simulink model "Drone_swarm_control"  (R2025a)
settings: Solver=FixedStepAuto  StartTime=0.0  StopTime=180  FixedStep=0.001  RelTol=1e-3
InitFcn:
  | %% Simulation parameters and waypoint trajectory
  | % Initial drone positions.
  | init_0=[0;0;0];
  | d_s=4;
  | init_1=init_0+d_s*[-1.1;0.1;0];
  | init_2=init_0+d_s*[0.3;-1.5;0];
  | init_3=init_0+d_s*[1.6;0.4;0];
  | init_4=init_0+d_s*[0.2;1.8;0];
  | 
  | % Initial battery energy in Wh.
  | E_0=77;
  | gain_2=1;
  | 
  | % PID controller gains.
  | PID_p=20;
  | PID_i=50;
  | PID_d=0;
  | 
  | % Router queues and background traffic.
  | router_buffer=160;
  | router_bandwith=300;
  | router_init_queue=[20,0,0,0,0];
  | traffic_mean=20;
  | traffic_variance=1;
  | 
  | % Communication-rate parameters.
  | F_max=2;
  | F_min=0.5;
  | F_H=(F_max+F_min)/3;
  | P_nc=(1-(F_H-F_min)/F_max);
  | 
  | 
  | % Desired formation offsets.
  | init_f_0=[0;0;0];
  | d_f=10;
  | init_f_1=init_0+d_f*[-1;0;0];
  | init_f_2=init_0+d_f*[0;-1;0];
  | init_f_3=init_0+d_f*[1;0;0];
  | init_f_4=init_0+d_f*[0;1;0];
  | 
  | 
  | % Waypoint mission with a fixed cruise altitude.
  | quota_fissa = -20;
  | 
  | waypoints = [
  |       0   0   0   0;
  |      75   0   quota_fissa   0;
  |     150   0   quota_fissa   0;
  |     225   0   quota_fissa   0;
  |     300   0   quota_fissa   0;
  |     300   0   quota_fissa   0;
  |     225  75   quota_fissa   0;
  |     150 150   quota_fissa   0;
  |      75 225   quota_fissa   0;
  |       0 300   quota_fissa   0;
  |       0 300   quota_fissa   0;
  |      75 300   quota_fissa   0;
  |     150 300   quota_fissa   0;
  |     225 300   quota_fissa   0;
  |     300 300   quota_fissa   0;
  | ... (+79 lines)
undefined symbols (not defined in the file): A_diacenza, DiscIntNeverNeededParam, L
libraries: dspsigops x10, robotcorelib x5, slpidlib x5, dspstat3 x5, simulink x1, uavutilslib x1
(part 3 of 4)

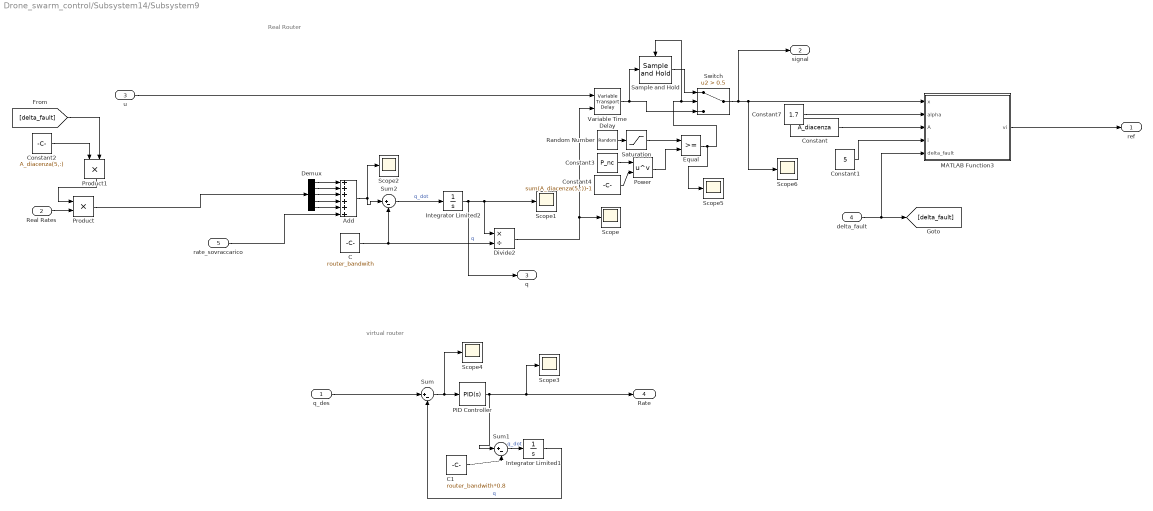
== system Drone_swarm_control/Subsystem14/Subsystem9 ==
  note: Real Router
  note: virtual router
  q_des : Inport
  " Real Rates" : Inport  Port=2
  u : Inport  Port=3
  delta_fault : Inport  Port=4
  "rate_sovraccarico " : Inport  Port=5
  Add : Sum  Inputs=++++++
  C : Constant  Value=router_bandwith
  C1 : Constant  Value=router_bandwith*0.8
  Constant : Constant  Value=A_diacenza
  Constant1 : Constant  Value=5
  Constant2 : Constant  Value=A_diacenza(5,:)
  Constant3 : Constant  Value=P_nc
  Constant4 : Constant  Value=sum(A_diacenza(5,:))-1
  Constant7 : Constant  Value=1.7
  Demux : Demux  Outputs=5
  Divide2 : Product  Inputs=*/
  Equal : RelationalOperator  OutDataTypeStr=boolean  RndMeth=Simplest  InputSameDT=off
  Integrator Limited1 : Integrator  InitialCondition=router_init_queue(1)  LimitOutput=on  UpperSaturationLimit=router_buffer  LowerSaturationLimit=0
  Integrator Limited2 : Integrator  InitialCondition=router_init_queue(5)  LimitOutput=on  UpperSaturationLimit=router_buffer  LowerSaturationLimit=0
  MATLAB Function3 : MATLAB Function  TreatAsAtomicUnit=on
  PID Controller : slpidlib/PID Controller  Controller=PID  Form=Parallel  TimeDomain=Continuous-time  UseExternalTs=off  SampleTime=-1  IntegratorMethod=Forward Euler  FilterMethod=Forward Euler  ControllerParametersSource=internal  P=PID_p  I=PID_i  UseKiTs=off  D=PID_d  UseExternalDerivativeSource=off  N=100  UseFilter=on  TunerSelectOption=Transfer Function Based (PID Tuner App)  InitialConditionSource=internal  InitialConditionForIntegrator=0  InitialConditionForFilter=0  DifferentiatorICPrevScaledInput=0  ExternalReset=none  TrackingMode=off  Kt=1  LimitOutput=off  SatLimitsSource=internal  UpperSaturationLimit=inf  LowerSaturationLimit=-inf  LinearizeAsGain=on  AntiWindupMode=none  Kb=1  LimitIntegrator=off  UpperIntegratorSaturationLimit=inf  LowerIntegratorSaturationLimit=-inf  POutMin=[]  POutMax=[]  IOutMin=[]  IOutMax=[]  DOutMin=[]  DOutMax=[]  NOutMin=[]  NOutMax=[]  SumOutMin=[]  SumOutMax=[]  SaturationOutMin=[]  SaturationOutMax=[]  PParamMin=[]  PParamMax=[]  IParamMin=[]  IParamMax=[]  DParamMin=[]  DParamMax=[]  NParamMin=[]  NParamMax=[]  KbParamMin=[]  KbParamMax=[]  KtParamMin=[]  KtParamMax=[]  KbOutMin=[]  KbOutMax=[]  KtOutMin=[]  KtOutMax=[]  IntegratorOutMin=[]  IntegratorOutMax=[]  FilterOutMin=[]  FilterOutMax=[]  SumI1OutMin=[]  SumI1OutMax=[]  SumI2OutMin=[]  SumI2OutMax=[]  SumI3OutMin=[]  SumI3OutMax=[]  SumI4OutMin=[]  SumI4OutMax=[]  SumDOutMin=[]  SumDOutMax=[]  DifferentiatorOutMin=[]  DifferentiatorOutMax=[]  FilterDiffOutCoefMin=[]  FilterDiffOutCoefMax=[]  ReciprocalOutMin=[]  ReciprocalOutMax=[]  SumDenOutMin=[]  SumDenOutMax=[]  SumNumOutMin=[]  SumNumOutMax=[]  DivideOutMin=[]  DivideOutMax=[]  UdiffTsProdOutMin=[]  UdiffTsProdOutMax=[]  NTsProdOutMin=[]  NTsProdOutMax=[]  UintegralTsProdOutMin=[]  UintegralTsProdOutMax=[]  UngainTsProdOutMin=[]  UngainTsProdOutMax=[]  ClampingZeroOutDataTypeStr=Inherit: Inherit via back propagation  ClampingZeroOutMin=[]  ClampingZeroOutMax=[]  FilterDenConstantOutDataTypeStr=Inherit: Inherit via back propagation  FilterDenConstantOutMin=[]  FilterDenConstantOutMax=[]  PCopyOutDataTypeStr=Inherit: Inherit via back propagation  PCopyOutMin=[]  PCopyOutMax=[]  NCopyOutDataTypeStr=Inherit: Inherit via back propagation  NCopyOutMin=[]  NCopyOutMax=[]  IntegratorContinuousStateAttributes=''  IntegratorStateMustResolveToSignalObject=off  IntegratorRTWStateStorageClass=Auto  FilterContinuousStateAttributes=''  FilterStateMustResolveToSignalObject=off  FilterRTWStateStorageClass=Auto  ParallelPVariant=InternalParameters  IdealPVariant=Disabled  IVariant=InternalParameters  DVariant=InternalParameters  IntegratorVariant=Continuous  SatVariant=Disabled  AWVariant=Passthrough  PCopyVariant=Disabled  TRVariant=Disabled  FdbkBlocksVariant=Forward  IdealPFdbkVariant=Disabled  SatFdbkVariant=Disabled  DerivativeFilterVariant=ContFilter  NVariant=InternalParameters  NCopyVariant=Disabled  FilterICVariant=InternalICsFilter  IntegratorICVariant=InternalICs  ExternalResetVariant=Disabled  TRSumVariant=Passthrough  SumFdbkVariant=Disabled  SumVariant=Sum_PID  TsampFilterVariant=InternalTs  TsampNgainVariant=Passthrough  TsampIntegralVariant=Disabled_SignalSpec  ExternalSaturationOutDataTypeStr=Inherit: Same as second input  DerivativeSourceVariant=ErrorSignal  PreIntVariant=InternalPreInt
  Power : Math  Operator=pow
  Product : Product
  Product1 : Product
  Random Number : RandomNumber  Mean=0.5  Variance=0.5  SampleTime=0.1
  Sample and Hold : dspsigops/Sample and Hold  trig=Rising edge  initCond=0  latchinput=off
  Saturation : Saturate  UpperLimit=1  LowerLimit=0
  Scope{,1..6} (7 alike) : Scope
      Scope settings: ActiveDisplayYMinimum=0.0019171133278549479  ActiveDisplayYMaximum=0.066506482659169808  DataLoggingVariableName=ScopeData7
      Scope1 settings: ActiveDisplayYMinimum=-1  ActiveDisplayYMaximum=1  DataLoggingVariableName=ScopeData8
      Scope2 settings: ActiveDisplayYMinimum=16.645701165470911  ActiveDisplayYMaximum=16.711897993083294  DataLoggingVariableName=ScopeData13
      Scope3 settings: ActiveDisplayYMinimum=-48.354575152001026  ActiveDisplayYMaximum=35.191176368009216  DataLoggingVariableName=ScopeData20
      Scope4 settings: ActiveDisplayYMinimum=-3.625  ActiveDisplayYMaximum=2.625  DataLoggingVariableName=ScopeData21
      Scope5 settings: ActiveDisplayYMinimum=-1  ActiveDisplayYMaximum=1  DataLoggingVariableName=ScopeData6
      Scope6 settings: ActiveDisplayYMinimum=-1  ActiveDisplayYMaximum=1  DataLoggingVariableName=ScopeData31
  Sum : Sum  Inputs=|+-
  Sum1 : Sum  Inputs=|+-
  Sum2 : Sum  Inputs=|+-
  Switch : Switch  Criteria=u2 > Threshold  Threshold=0.5  SaturateOnIntegerOverflow=off  InputSameDT=off
  Variable Time Delay : VariableTransportDelay  MaximumDelay=1000  InitialOutput=[init_0;zeros(6,1);init_1;zeros(6,1);init_2;zeros(6,1);init_3;zeros(6,1);init_4;zeros(6,1);]  MaximumPoints=1e4  ZeroDelay=on
  ref : Outport
  "signal " : Outport  Port=2
  q : Outport  Port=3
  " Rate" : Outport  Port=4
  wires:
  Constant7/1 -> MATLAB Function3/2(alpha)
  Constant/1 -> MATLAB Function3/3(A)
  Constant1/1 -> MATLAB Function3/4(i)
  MATLAB Function3/1(vi) -> ref/1
  Integrator Limited2/1 -> Scope1/1, Divide2/1, q/1  "q"
  Switch/1 -> "signal "/1, Scope6/1, MATLAB Function3/1(x)
  u/1 -> Variable Time Delay/1
  Sum2/1 -> Integrator Limited2/1  "q_dot"
  Divide2/1 -> Scope/1, Variable Time Delay/2
  C/1 -> Divide2/2, Sum2/2
  Sample and Hold/1 -> Switch/1
  Add/1 -> Sum2/1, Scope2/1
  Integrator Limited1/1 -> Sum/2  "q"
  PID Controller/1 -> Sum1/1, " Rate"/1, Scope3/1
  Sum1/1 -> Integrator Limited1/1  "q_dot"
  C1/1 -> Sum1/2
  Sum/1 -> Scope4/1, PID Controller/1
  q_des/1 -> Sum/1
  Demux/1 -> Add/1
  Demux/2 -> Add/2
  Demux/3 -> Add/3
  Demux/4 -> Add/4
  Demux/5 -> Add/5
  Power/1 -> Equal/2
  Saturation/1 -> Equal/1
  Random Number/1 -> Saturation/1
  Constant4/1 -> Power/2
  Equal/1 -> Scope5/1, Sample and Hold/Trigger, Switch/2
  Constant3/1 -> Power/1
  Variable Time Delay/1 -> Sample and Hold/1, Switch/3
  delta_fault/1 -> [delta_fault], MATLAB Function3/5(delta_fault)
  Product1/1 -> Product/1
  [delta_fault] -> Product1/2
  Constant2/1 -> Product1/1
  " Real Rates"/1 -> Product/2
  Product/1 -> Demux/1
  "rate_sovraccarico "/1 -> Add/6

== system Drone_swarm_control/Subsystem5/Subsystem ==
  output : Inport
  Cast To Double : DataTypeConversion  OutDataTypeStr=double  SaturateOnIntegerOverflow=off  RndMeth=Floor
  Constant : Constant  Value=5
  Constant1 : Constant
  Detect Rise Positive : simulink/Logic and Bit Operations/Detect Rise Positive  vinit=0  OutDataTypeStr=boolean
  Gain : Gain  Gain=1e5
  Integrator : Integrator  ExternalReset=rising
  Saturation : Saturate  UpperLimit=1  LowerLimit=0
  Scope{,1..3} (4 alike) : Scope
      Scope settings: ActiveDisplayYMinimum=-0.12499999999999997  ActiveDisplayYMaximum=1.125  DataLoggingVariableName=ScopeData46
      Scope1 settings: ActiveDisplayYMinimum=-1  ActiveDisplayYMaximum=1  DataLoggingVariableName=ScopeData47
      Scope2 settings: ActiveDisplayYMinimum=-0.00012499999999999998  ActiveDisplayYMaximum=0.0011250000000000001  DataLoggingVariableName=ScopeData48
      Scope3 settings: DataLoggingVariableName=ScopeData49
  Variable Transport Delay : VariableTransportDelay  MaximumDelay=10
  Variable Transport Delay1 : VariableTransportDelay  MaximumDelay=10
  Out1 : Outport
  wires:
  Variable Transport Delay/1 -> Scope1/1, Integrator/2
  Cast To Double/1 -> Integrator/1, Variable Transport Delay/1
  Integrator/1 -> Scope2/1, Gain/1
  Constant/1 -> Variable Transport Delay/2
  Saturation/1 -> Scope3/1, Out1/1
  output/1 -> Variable Transport Delay1/1
  Gain/1 -> Saturation/1
  Detect Rise Positive/1 -> Scope/1, Cast To Double/1
  Variable Transport Delay1/1 -> Detect Rise Positive/1
  Constant1/1 -> Variable Transport Delay1/2

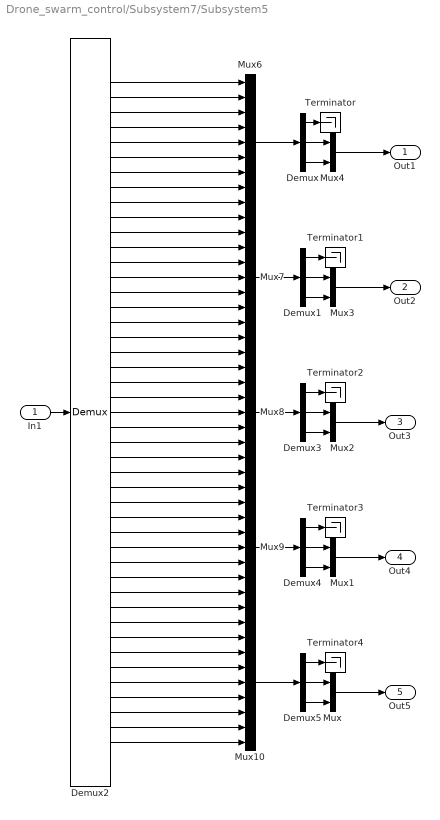
== system Drone_swarm_control/Subsystem7/Subsystem5 ==
  In1 : Inport
  Demux{,1,3..5} (5 alike) : Demux  Outputs=3
  Demux2 : Demux  Outputs=45
  Mux{,1..4} (5 alike) : Mux  Inputs=2
  Mux{6..10} (5 alike) : Mux  Inputs=9
  Terminator{,1..4} (5 alike) : Terminator
  Out1 : Outport
  Out2 : Outport  Port=2
  Out3 : Outport  Port=3
  Out4 : Outport  Port=4
  Out5 : Outport  Port=5
  wires:
  Demux2/4 -> Mux6/4
  Demux2/22 -> Mux8/4
  Demux2/7 -> Mux6/7
  Demux2/5 -> Mux6/5
  Demux2/37 -> Mux10/1
  Demux2/32 -> Mux9/5
  Demux2/11 -> Mux7/2
  Demux2/35 -> Mux9/8
  Demux2/39 -> Mux10/3
  Demux2/12 -> Mux7/3
  Demux2/9 -> Mux6/9
  Demux2/18 -> Mux7/9
  Demux2/25 -> Mux8/7
  Demux2/6 -> Mux6/6
  Demux2/31 -> Mux9/4
  Demux2/42 -> Mux10/6
  Demux2/1 -> Mux6/1
  Demux2/17 -> Mux7/8
  Demux2/29 -> Mux9/2
  Demux2/24 -> Mux8/6
  Demux2/8 -> Mux6/8
  Demux2/28 -> Mux9/1
  Demux2/45 -> Mux10/9
  Demux2/44 -> Mux10/8
  Demux2/16 -> Mux7/7
  Demux2/38 -> Mux10/2
  Demux2/21 -> Mux8/3
  Demux2/19 -> Mux8/1
  Demux2/33 -> Mux9/6
  Demux2/36 -> Mux9/9
  Demux2/23 -> Mux8/5
  Demux2/43 -> Mux10/7
  Demux2/30 -> Mux9/3
  Demux2/41 -> Mux10/5
  Demux2/34 -> Mux9/7
  Demux2/14 -> Mux7/5
  Demux2/15 -> Mux7/6
  Demux2/3 -> Mux6/3
  Demux2/13 -> Mux7/4
  Demux2/26 -> Mux8/8
  Demux2/20 -> Mux8/2
  Demux2/2 -> Mux6/2
  Demux2/27 -> Mux8/9
  Demux2/10 -> Mux7/1
  Demux2/40 -> Mux10/4
  In1/1 -> Demux2/1
  Mux6/1 -> Demux/1
  Mux7/1 -> Demux1/1
  Mux8/1 -> Demux3/1
  Mux9/1 -> Demux4/1
  Mux10/1 -> Demux5/1
  Demux/1 -> Terminator/1
  Demux1/1 -> Terminator1/1
  Demux3/1 -> Terminator2/1
  Demux4/1 -> Terminator3/1
  Demux5/1 -> Terminator4/1
  Demux5/3 -> Mux/2
  Demux5/2 -> Mux/1
  Mux/1 -> Out5/1
  Demux4/2 -> Mux1/1
  Demux4/3 -> Mux1/2
  Mux1/1 -> Out4/1
  Demux3/2 -> Mux2/1
  Demux3/3 -> Mux2/2
  Mux2/1 -> Out3/1
  Demux1/2 -> Mux3/1
  Demux1/3 -> Mux3/2
  Mux3/1 -> Out2/1
  Demux/2 -> Mux4/1
  Demux/3 -> Mux4/2
  Mux4/1 -> Out1/1

== system Drone_swarm_control/trasmission/Subsystem1 ==
  note: Subsystem13
  In : Inport
  In1 : Inport  Port=2
  Constant13 : Constant
  Constant2 : Constant
  Divide : Product  Inputs=*/
  Integrator : Integrator  ExternalReset=rising
  Relational Operator : RelationalOperator  Operator=<=  OutDataTypeStr=boolean  RndMeth=Simplest  InputSameDT=off
  Sample and Hold5 : dspsigops/Sample and Hold  trig=Rising edge  initCond=0  latchinput=off
  Scope3 : Scope
      settings: ActiveDisplayYMinimum=-3.131696080231905E+7  ActiveDisplayYMaximum=3.596063759040764E+7  DataLoggingVariableName=ScopeData9
  Switch : Switch  Criteria=u2 > Threshold  SaturateOnIntegerOverflow=off  InputSameDT=off
  Unit Delay : UnitDelay  SampleTime=Ts  HasFrameUpgradeWarning=on
  " " : Outport
  wires:
  In/1 -> Sample and Hold5/1
  Constant2/1 -> Integrator/1
  In1/1 -> Divide/2
  Unit Delay/1 -> Integrator/2
  Constant13/1 -> Divide/1
  Divide/1 -> Relational Operator/1, Scope3/1
  Relational Operator/1 -> Unit Delay/1, Sample and Hold5/Trigger
  Sample and Hold5/1 -> " "/1
  Integrator/1 -> Relational Operator/2

== system Drone_swarm_control/trasmission/Subsystem2 ==
  note: Subsystem13
  In : Inport
  In1 : Inport  Port=2
  Constant13 : Constant
  Constant2 : Constant
  Divide : Product  Inputs=*/
  Integrator : Integrator  ExternalReset=rising
  Relational Operator : RelationalOperator  Operator=<=  OutDataTypeStr=boolean  RndMeth=Simplest  InputSameDT=off
  Sample and Hold5 : dspsigops/Sample and Hold  trig=Rising edge  initCond=0  latchinput=off
  Scope3 : Scope
      settings: ActiveDisplayYMinimum=-3.131696080231905E+7  ActiveDisplayYMaximum=3.596063759040764E+7  DataLoggingVariableName=ScopeData9
  Unit Delay : UnitDelay  SampleTime=Ts  HasFrameUpgradeWarning=on
  " " : Outport
  wires:
  In/1 -> Sample and Hold5/1
  Constant2/1 -> Integrator/1
  In1/1 -> Divide/2
  Unit Delay/1 -> Integrator/2
  Constant13/1 -> Divide/1
  Divide/1 -> Relational Operator/1, Scope3/1
  Relational Operator/1 -> Unit Delay/1, Sample and Hold5/Trigger
  Sample and Hold5/1 -> " "/1
  Integrator/1 -> Relational Operator/2

== system Drone_swarm_control/trasmission/Subsystem3 ==
  note: Subsystem13
  In : Inport
  In1 : Inport  Port=2
  Constant13 : Constant
  Constant2 : Constant
  Divide : Product  Inputs=*/
  Integrator : Integrator  ExternalReset=rising
  Relational Operator : RelationalOperator  Operator=<=  OutDataTypeStr=boolean  RndMeth=Simplest  InputSameDT=off
  Sample and Hold5 : dspsigops/Sample and Hold  trig=Rising edge  initCond=0  latchinput=off
  Scope3 : Scope
      settings: ActiveDisplayYMinimum=-3.131696080231905E+7  ActiveDisplayYMaximum=3.596063759040764E+7  DataLoggingVariableName=ScopeData9
  Unit Delay : UnitDelay  SampleTime=Ts  HasFrameUpgradeWarning=on
  " " : Outport
  wires:
  Integrator/1 -> Relational Operator/2
  Sample and Hold5/1 -> " "/1
  Relational Operator/1 -> Sample and Hold5/Trigger, Unit Delay/1
  Divide/1 -> Scope3/1, Relational Operator/1
  Constant13/1 -> Divide/1
  Unit Delay/1 -> Integrator/2
  In1/1 -> Divide/2
  Constant2/1 -> Integrator/1
  In/1 -> Sample and Hold5/1

== system Drone_swarm_control/trasmission/Subsystem4 ==
  note: Subsystem13
  In : Inport
  In1 : Inport  Port=2
  Constant13 : Constant
  Constant2 : Constant
  Divide : Product  Inputs=*/
  Integrator : Integrator  ExternalReset=rising
  Relational Operator : RelationalOperator  Operator=<=  OutDataTypeStr=boolean  RndMeth=Simplest  InputSameDT=off
  Sample and Hold5 : dspsigops/Sample and Hold  trig=Rising edge  initCond=0  latchinput=off
  Scope3 : Scope
      settings: ActiveDisplayYMinimum=-3.131696080231905E+7  ActiveDisplayYMaximum=3.596063759040764E+7  DataLoggingVariableName=ScopeData9
  Unit Delay : UnitDelay  SampleTime=Ts  HasFrameUpgradeWarning=on
  " " : Outport
  wires:
  In/1 -> Sample and Hold5/1
  Constant2/1 -> Integrator/1
  In1/1 -> Divide/2
  Unit Delay/1 -> Integrator/2
  Constant13/1 -> Divide/1
  Divide/1 -> Relational Operator/1, Scope3/1
  Relational Operator/1 -> Unit Delay/1, Sample and Hold5/Trigger
  Sample and Hold5/1 -> " "/1
  Integrator/1 -> Relational Operator/2

== system Drone_swarm_control/trasmission/Subsystem5 ==
  note: Subsystem13
  In : Inport
  In1 : Inport  Port=2
  Constant13 : Constant
  Constant2 : Constant
  Divide : Product  Inputs=*/
  Integrator : Integrator  ExternalReset=rising
  Relational Operator : RelationalOperator  Operator=<=  OutDataTypeStr=boolean  RndMeth=Simplest  InputSameDT=off
  Sample and Hold5 : dspsigops/Sample and Hold  trig=Rising edge  initCond=0  latchinput=off
  Scope3 : Scope
      settings: ActiveDisplayYMinimum=-3.131696080231905E+7  ActiveDisplayYMaximum=3.596063759040764E+7  DataLoggingVariableName=ScopeData9
  Unit Delay : UnitDelay  SampleTime=Ts  HasFrameUpgradeWarning=on
  " " : Outport
  wires:
  Integrator/1 -> Relational Operator/2
  Sample and Hold5/1 -> " "/1
  Relational Operator/1 -> Sample and Hold5/Trigger, Unit Delay/1
  Divide/1 -> Scope3/1, Relational Operator/1
  Constant13/1 -> Divide/1
  Unit Delay/1 -> Integrator/2
  In1/1 -> Divide/2
  Constant2/1 -> Integrator/1
  In/1 -> Sample and Hold5/1

== system Drone_swarm_control/trasmission/rate_min ==
  r_req : Inport
  delta_fault : Inport  Port=2
  Constant : Constant  Value=A_diacenza
  MATLAB Function : MATLAB Function  TreatAsAtomicUnit=on
  MATLAB Function1 : MATLAB Function  TreatAsAtomicUnit=on
  MATLAB Function2 : MATLAB Function  TreatAsAtomicUnit=on
  MATLAB Function3 : MATLAB Function  TreatAsAtomicUnit=on
  MATLAB Function4 : MATLAB Function  TreatAsAtomicUnit=on
  MATLAB Function5 : MATLAB Function  TreatAsAtomicUnit=on
  Minimum{,1..4} (5 alike) : dspstat3/Minimum  operation=minimum  fcn=Value  indexBase=One  operateOver=Each column  Dimension=1  InputProcessing=Columns as channels (frame based)  reset=None  roiEnable=off  roiType=Rectangles  roiPortion=Entire ROI  roiOutput=Individual statistics for each ROI  roiFlag=off  roundingMode=Floor  overflowMode=off
      settings: LibrarySourceBlock=dsphdlsupportstat/Minimum
  Mux1 : Mux  Inputs=5
  Product{,1..4} (5 alike) : Product
  r_min : Outport
  wires:
  MATLAB Function/1(y) -> Minimum/1
  Minimum3/1 -> Mux1/4
  Mux1/1 -> r_min/1
  MATLAB Function4/1(y) -> Minimum4/1
  Minimum2/1 -> Mux1/3
  Minimum4/1 -> Mux1/5
  MATLAB Function2/1(y) -> Minimum2/1
  MATLAB Function1/1(y) -> Minimum1/1
  Minimum/1 -> Mux1/1
  Minimum1/1 -> Mux1/2
  MATLAB Function3/1(y) -> Minimum3/1
  delta_fault/1 -> MATLAB Function5/2(delta)
  Constant/1 -> MATLAB Function5/1(A)
  Product/1 -> MATLAB Function/1(u)
  Product1/1 -> MATLAB Function1/1(u)
  Product2/1 -> MATLAB Function2/1(u)
  Product3/1 -> MATLAB Function3/1(u)
  Product4/1 -> MATLAB Function4/1(u)
  r_req/1 -> Product1/2, Product/2, Product4/2, Product3/2, Product2/2
  MATLAB Function5/1(A_edit1) -> Product/1
  MATLAB Function5/2(A_edit2) -> Product1/1
  MATLAB Function5/3(A_edit3) -> Product2/1
  MATLAB Function5/4(A_edit4) -> Product3/1
  MATLAB Function5/5(A_edit5) -> Product4/1

== system Drone_swarm_control/Subsystem1/Subsystem_1/Inner-loop control ==
  zb_des : Inport
  Rb : Inport  Port=2
  omega_bb : Inport  Port=3
  xb_des : Inport  Port=4
  Derivation : DiscreteTransferFcn  Numerator=[1 -1]  Denominator=[Ts 0]  InitialStates=[1 0 0;0 1 0;0 0 1]  SampleTime=Ts
  Derivation1 : DiscreteTransferFcn  Numerator=[1 -1]  Denominator=[Ts 0]  InitialStates=[0 0 0]  SampleTime=Ts
  Inner-loop control : MATLAB Function  TreatAsAtomicUnit=on
  Unit Delay1 : UnitDelay  InitialCondition=eye(3)  SampleTime=Ts
  Unit Delay3 : UnitDelay  InitialCondition=[0 0 0]  SampleTime=Ts
  tau : Outport
  err_R : Outport  Port=2
  err_W : Outport  Port=3
  wires:
  Inner-loop control/2(omega_bb_des) -> Derivation1/1
  Inner-loop control/1(Rb_des) -> Derivation/1
  omega_bb/1 -> Inner-loop control/4(omega_bb)
  zb_des/1 -> Inner-loop control/1(zb_des)
  Derivation/1 -> Unit Delay1/1
  Unit Delay3/1 -> Inner-loop control/5(dot_omega_bb_des)
  Inner-loop control/5(err_W) -> err_W/1
  Derivation1/1 -> Unit Delay3/1
  Unit Delay1/1 -> Inner-loop control/3(dot_Rb_des)
  Inner-loop control/3(tau) -> tau/1
  Rb/1 -> Inner-loop control/2(Rb)
  Inner-loop control/4(err_R) -> err_R/1
  xb_des/1 -> Inner-loop control/6(xb_des)

== system Drone_swarm_control/Subsystem1/Subsystem_1/Planner ==
  References : Inport
  Constant : Constant  Value=0
  Demux : Demux  Outputs=10
  Mux{1..4} (4 alike) : Mux  Inputs=3
  Trigonometric Function : Trigonometry
  Trigonometric Function1 : Trigonometry  Operator=cos
  position_des : Outport
  linear_velocity_des : Outport  Port=2
  linear_acceleration_des : Outport  Port=3
  xb_des : Outport  Port=4
  wires:
  References/1 -> Demux/1
  Demux/10 -> Trigonometric Function1/1, Trigonometric Function/1
  Demux/9 -> Mux1/3
  Demux/8 -> Mux1/2
  Demux/7 -> Mux1/1
  Demux/6 -> Mux3/3
  Demux/5 -> Mux3/2
  Demux/4 -> Mux3/1
  Demux/3 -> Mux2/3
  Demux/2 -> Mux2/2
  Demux/1 -> Mux2/1
  Constant/1 -> Mux4/3
  Trigonometric Function1/1 -> Mux4/1
  Trigonometric Function/1 -> Mux4/2
  Mux4/1 -> xb_des/1
  Mux2/1 -> position_des/1
  Mux3/1 -> linear_velocity_des/1
  Mux1/1 -> linear_acceleration_des/1

== system Drone_swarm_control/Subsystem1/Subsystem_1/Quadrotor dynamics ==
  uT : Inport
  tau_b : Inport  Port=2
  Integrator : Integrator  InitialCondition=init_0
  Integrator1 : Integrator  InitialCondition=lin_vel_0
  Integrator2 : Integrator  InitialCondition=[1 0 0; 0 1 0;0 0 1]
  Integrator3 : Integrator  InitialCondition=w_bb_0
  MATLAB Function1 : MATLAB Function  TreatAsAtomicUnit=on
  UAV dynamics : MATLAB Function  TreatAsAtomicUnit=on
  Position : Outport
  Linear_velocity : Outport  Port=2
  Rb : Outport  Port=3
  dot_Rb : Outport  Port=4
  omega_bb : Outport  Port=5
  dot_omega_bb : Outport  Port=6
  lin_acc : Outport  Port=7
  wires:
  Integrator2/1 -> MATLAB Function1/1(Rb_temp)
  MATLAB Function1/1(Rb) -> UAV dynamics/3(Rb), Rb/1
  UAV dynamics/2(dot_Rb) -> dot_Rb/1, Integrator2/1
  Integrator3/1 -> UAV dynamics/4(omega_bb), omega_bb/1
  Integrator1/1 -> Integrator/1, Linear_velocity/1
  uT/1 -> UAV dynamics/1(uT)
  UAV dynamics/1(lin_acc) -> Integrator1/1, lin_acc/1
  UAV dynamics/3(ang_acc) -> Integrator3/1, dot_omega_bb/1
  Integrator/1 -> Position/1
  tau_b/1 -> UAV dynamics/2(tau_b)

== system Drone_swarm_control/Subsystem1/Subsystem_2/Inner-loop control ==
  zb_des : Inport
  Rb : Inport  Port=2
  omega_bb : Inport  Port=3
  xb_des : Inport  Port=4
  Derivation : DiscreteTransferFcn  Numerator=[1 -1]  Denominator=[Ts 0]  InitialStates=[1 0 0;0 1 0;0 0 1]  SampleTime=Ts
  Derivation1 : DiscreteTransferFcn  Numerator=[1 -1]  Denominator=[Ts 0]  InitialStates=[0 0 0]  SampleTime=Ts
  Inner-loop control : MATLAB Function  TreatAsAtomicUnit=on
  Unit Delay1 : UnitDelay  InitialCondition=eye(3)  SampleTime=Ts
  Unit Delay3 : UnitDelay  InitialCondition=[0 0 0]  SampleTime=Ts
  tau : Outport
  err_R : Outport  Port=2
  err_W : Outport  Port=3
  wires:
  Inner-loop control/2(omega_bb_des) -> Derivation1/1
  Inner-loop control/1(Rb_des) -> Derivation/1
  omega_bb/1 -> Inner-loop control/4(omega_bb)
  zb_des/1 -> Inner-loop control/1(zb_des)
  Derivation/1 -> Unit Delay1/1
  Unit Delay3/1 -> Inner-loop control/5(dot_omega_bb_des)
  Inner-loop control/5(err_W) -> err_W/1
  Derivation1/1 -> Unit Delay3/1
  Unit Delay1/1 -> Inner-loop control/3(dot_Rb_des)
  Inner-loop control/3(tau) -> tau/1
  Rb/1 -> Inner-loop control/2(Rb)
  Inner-loop control/4(err_R) -> err_R/1
  xb_des/1 -> Inner-loop control/6(xb_des)

== system Drone_swarm_control/Subsystem1/Subsystem_2/Planner ==
  References : Inport
  Constant : Constant  Value=0
  Demux : Demux  Outputs=10
  Mux{1..4} (4 alike) : Mux  Inputs=3
  Trigonometric Function : Trigonometry
  Trigonometric Function1 : Trigonometry  Operator=cos
  position_des : Outport
  linear_velocity_des : Outport  Port=2
  linear_acceleration_des : Outport  Port=3
  xb_des : Outport  Port=4
  wires:
  References/1 -> Demux/1
  Demux/10 -> Trigonometric Function1/1, Trigonometric Function/1
  Demux/9 -> Mux1/3
  Demux/8 -> Mux1/2
  Demux/7 -> Mux1/1
  Demux/6 -> Mux3/3
  Demux/5 -> Mux3/2
  Demux/4 -> Mux3/1
  Demux/3 -> Mux2/3
  Demux/2 -> Mux2/2
  Demux/1 -> Mux2/1
  Constant/1 -> Mux4/3
  Trigonometric Function1/1 -> Mux4/1
  Trigonometric Function/1 -> Mux4/2
  Mux4/1 -> xb_des/1
  Mux2/1 -> position_des/1
  Mux3/1 -> linear_velocity_des/1
  Mux1/1 -> linear_acceleration_des/1

== system Drone_swarm_control/Subsystem1/Subsystem_2/Quadrotor dynamics ==
  uT : Inport
  tau_b : Inport  Port=2
  Integrator : Integrator  InitialCondition=init_1
  Integrator1 : Integrator  InitialCondition=lin_vel_0
  Integrator2 : Integrator  InitialCondition=[1 0 0; 0 1 0;0 0 1]
  Integrator3 : Integrator  InitialCondition=w_bb_0
  MATLAB Function1 : MATLAB Function  TreatAsAtomicUnit=on
  UAV dynamics : MATLAB Function  TreatAsAtomicUnit=on
  Position : Outport
  Linear_velocity : Outport  Port=2
  Rb : Outport  Port=3
  dot_Rb : Outport  Port=4
  omega_bb : Outport  Port=5
  dot_omega_bb : Outport  Port=6
  lin_acc : Outport  Port=7
  wires:
  Integrator2/1 -> MATLAB Function1/1(Rb_temp)
  MATLAB Function1/1(Rb) -> UAV dynamics/3(Rb), Rb/1
  UAV dynamics/2(dot_Rb) -> dot_Rb/1, Integrator2/1
  Integrator3/1 -> omega_bb/1, UAV dynamics/4(omega_bb)
  Integrator1/1 -> Integrator/1, Linear_velocity/1
  uT/1 -> UAV dynamics/1(uT)
  UAV dynamics/1(lin_acc) -> Integrator1/1, lin_acc/1
  UAV dynamics/3(ang_acc) -> Integrator3/1, dot_omega_bb/1
  Integrator/1 -> Position/1
  tau_b/1 -> UAV dynamics/2(tau_b)

== system Drone_swarm_control/Subsystem1/Subsystem_3/Inner-loop control ==
  zb_des : Inport
  Rb : Inport  Port=2
  omega_bb : Inport  Port=3
  xb_des : Inport  Port=4
  Derivation : DiscreteTransferFcn  Numerator=[1 -1]  Denominator=[Ts 0]  InitialStates=[1 0 0;0 1 0;0 0 1]  SampleTime=Ts
  Derivation1 : DiscreteTransferFcn  Numerator=[1 -1]  Denominator=[Ts 0]  InitialStates=[0 0 0]  SampleTime=Ts
  Inner-loop control : MATLAB Function  TreatAsAtomicUnit=on
  Unit Delay1 : UnitDelay  InitialCondition=eye(3)  SampleTime=Ts
  Unit Delay3 : UnitDelay  InitialCondition=[0 0 0]  SampleTime=Ts
  tau : Outport
  err_R : Outport  Port=2
  err_W : Outport  Port=3
  wires:
  Inner-loop control/2(omega_bb_des) -> Derivation1/1
  Inner-loop control/1(Rb_des) -> Derivation/1
  omega_bb/1 -> Inner-loop control/4(omega_bb)
  zb_des/1 -> Inner-loop control/1(zb_des)
  Derivation/1 -> Unit Delay1/1
  Unit Delay3/1 -> Inner-loop control/5(dot_omega_bb_des)
  Inner-loop control/5(err_W) -> err_W/1
  Derivation1/1 -> Unit Delay3/1
  Unit Delay1/1 -> Inner-loop control/3(dot_Rb_des)
  Inner-loop control/3(tau) -> tau/1
  Rb/1 -> Inner-loop control/2(Rb)
  Inner-loop control/4(err_R) -> err_R/1
  xb_des/1 -> Inner-loop control/6(xb_des)

== system Drone_swarm_control/Subsystem1/Subsystem_3/Planner ==
  References : Inport
  Constant : Constant  Value=0
  Demux : Demux  Outputs=10
  Mux{1..4} (4 alike) : Mux  Inputs=3
  Trigonometric Function : Trigonometry
  Trigonometric Function1 : Trigonometry  Operator=cos
  position_des : Outport
  linear_velocity_des : Outport  Port=2
  linear_acceleration_des : Outport  Port=3
  xb_des : Outport  Port=4
  wires:
  References/1 -> Demux/1
  Demux/10 -> Trigonometric Function1/1, Trigonometric Function/1
  Demux/9 -> Mux1/3
  Demux/8 -> Mux1/2
  Demux/7 -> Mux1/1
  Demux/6 -> Mux3/3
  Demux/5 -> Mux3/2
  Demux/4 -> Mux3/1
  Demux/3 -> Mux2/3
  Demux/2 -> Mux2/2
  Demux/1 -> Mux2/1
  Constant/1 -> Mux4/3
  Trigonometric Function1/1 -> Mux4/1
  Trigonometric Function/1 -> Mux4/2
  Mux4/1 -> xb_des/1
  Mux2/1 -> position_des/1
  Mux3/1 -> linear_velocity_des/1
  Mux1/1 -> linear_acceleration_des/1

== system Drone_swarm_control/Subsystem1/Subsystem_3/Quadrotor dynamics ==
  uT : Inport
  tau_b : Inport  Port=2
  Integrator : Integrator  InitialCondition=init_2
  Integrator1 : Integrator  InitialCondition=lin_vel_0
  Integrator2 : Integrator  InitialCondition=[1 0 0; 0 1 0;0 0 1]
  Integrator3 : Integrator  InitialCondition=w_bb_0
  MATLAB Function1 : MATLAB Function  TreatAsAtomicUnit=on
  UAV dynamics : MATLAB Function  TreatAsAtomicUnit=on
  Position : Outport
  Linear_velocity : Outport  Port=2
  Rb : Outport  Port=3
  dot_Rb : Outport  Port=4
  omega_bb : Outport  Port=5
  dot_omega_bb : Outport  Port=6
  lin_acc : Outport  Port=7
  wires:
  Integrator2/1 -> MATLAB Function1/1(Rb_temp)
  MATLAB Function1/1(Rb) -> UAV dynamics/3(Rb), Rb/1
  UAV dynamics/2(dot_Rb) -> dot_Rb/1, Integrator2/1
  Integrator3/1 -> omega_bb/1, UAV dynamics/4(omega_bb)
  Integrator1/1 -> Integrator/1, Linear_velocity/1
  uT/1 -> UAV dynamics/1(uT)
  UAV dynamics/1(lin_acc) -> Integrator1/1, lin_acc/1
  UAV dynamics/3(ang_acc) -> Integrator3/1, dot_omega_bb/1
  Integrator/1 -> Position/1
  tau_b/1 -> UAV dynamics/2(tau_b)

== system Drone_swarm_control/Subsystem1/Subsystem_4/Inner-loop control ==
  zb_des : Inport
  Rb : Inport  Port=2
  omega_bb : Inport  Port=3
  xb_des : Inport  Port=4
  Derivation : DiscreteTransferFcn  Numerator=[1 -1]  Denominator=[Ts 0]  InitialStates=[1 0 0;0 1 0;0 0 1]  SampleTime=Ts
  Derivation1 : DiscreteTransferFcn  Numerator=[1 -1]  Denominator=[Ts 0]  InitialStates=[0 0 0]  SampleTime=Ts
  Inner-loop control : MATLAB Function  TreatAsAtomicUnit=on
  Unit Delay1 : UnitDelay  InitialCondition=eye(3)  SampleTime=Ts
  Unit Delay3 : UnitDelay  InitialCondition=[0 0 0]  SampleTime=Ts
  tau : Outport
  err_R : Outport  Port=2
  err_W : Outport  Port=3
  wires:
  Inner-loop control/2(omega_bb_des) -> Derivation1/1
  Inner-loop control/1(Rb_des) -> Derivation/1
  omega_bb/1 -> Inner-loop control/4(omega_bb)
  zb_des/1 -> Inner-loop control/1(zb_des)
  Derivation/1 -> Unit Delay1/1
  Unit Delay3/1 -> Inner-loop control/5(dot_omega_bb_des)
  Inner-loop control/5(err_W) -> err_W/1
  Derivation1/1 -> Unit Delay3/1
  Unit Delay1/1 -> Inner-loop control/3(dot_Rb_des)
  Inner-loop control/3(tau) -> tau/1
  Rb/1 -> Inner-loop control/2(Rb)
  Inner-loop control/4(err_R) -> err_R/1
  xb_des/1 -> Inner-loop control/6(xb_des)

== system Drone_swarm_control/Subsystem1/Subsystem_4/Planner ==
  References : Inport
  Constant : Constant  Value=0
  Demux : Demux  Outputs=10
  Mux{1..4} (4 alike) : Mux  Inputs=3
  Trigonometric Function : Trigonometry
  Trigonometric Function1 : Trigonometry  Operator=cos
  position_des : Outport
  linear_velocity_des : Outport  Port=2
  linear_acceleration_des : Outport  Port=3
  xb_des : Outport  Port=4
  wires:
  References/1 -> Demux/1
  Demux/10 -> Trigonometric Function1/1, Trigonometric Function/1
  Demux/9 -> Mux1/3
  Demux/8 -> Mux1/2
  Demux/7 -> Mux1/1
  Demux/6 -> Mux3/3
  Demux/5 -> Mux3/2
  Demux/4 -> Mux3/1
  Demux/3 -> Mux2/3
  Demux/2 -> Mux2/2
  Demux/1 -> Mux2/1
  Constant/1 -> Mux4/3
  Trigonometric Function1/1 -> Mux4/1
  Trigonometric Function/1 -> Mux4/2
  Mux4/1 -> xb_des/1
  Mux2/1 -> position_des/1
  Mux1/1 -> linear_acceleration_des/1
  Mux3/1 -> linear_velocity_des/1

== system Drone_swarm_control/Subsystem1/Subsystem_4/Quadrotor dynamics ==
  uT : Inport
  tau_b : Inport  Port=2
  Integrator : Integrator  InitialCondition=init_3
  Integrator1 : Integrator  InitialCondition=lin_vel_0
  Integrator2 : Integrator  InitialCondition=[1 0 0; 0 1 0;0 0 1]
  Integrator3 : Integrator  InitialCondition=w_bb_0
  MATLAB Function1 : MATLAB Function  TreatAsAtomicUnit=on
  UAV dynamics : MATLAB Function  TreatAsAtomicUnit=on
  Position : Outport
  Linear_velocity : Outport  Port=2
  Rb : Outport  Port=3
  dot_Rb : Outport  Port=4
  omega_bb : Outport  Port=5
  dot_omega_bb : Outport  Port=6
  lin_acc : Outport  Port=7
  wires:
  Integrator2/1 -> MATLAB Function1/1(Rb_temp)
  MATLAB Function1/1(Rb) -> UAV dynamics/3(Rb), Rb/1
  UAV dynamics/2(dot_Rb) -> dot_Rb/1, Integrator2/1
  Integrator3/1 -> omega_bb/1, UAV dynamics/4(omega_bb)
  Integrator1/1 -> Integrator/1, Linear_velocity/1
  uT/1 -> UAV dynamics/1(uT)
  UAV dynamics/1(lin_acc) -> Integrator1/1, lin_acc/1
  UAV dynamics/3(ang_acc) -> Integrator3/1, dot_omega_bb/1
  Integrator/1 -> Position/1
  tau_b/1 -> UAV dynamics/2(tau_b)

== system Drone_swarm_control/Subsystem1/Subsystem_5/Inner-loop control ==
  zb_des : Inport
  Rb : Inport  Port=2
  omega_bb : Inport  Port=3
  xb_des : Inport  Port=4
  Derivation : DiscreteTransferFcn  Numerator=[1 -1]  Denominator=[Ts 0]  InitialStates=[1 0 0;0 1 0;0 0 1]  SampleTime=Ts
  Derivation1 : DiscreteTransferFcn  Numerator=[1 -1]  Denominator=[Ts 0]  InitialStates=[0 0 0]  SampleTime=Ts
  Inner-loop control : MATLAB Function  TreatAsAtomicUnit=on
  Unit Delay1 : UnitDelay  InitialCondition=eye(3)  SampleTime=Ts
  Unit Delay3 : UnitDelay  InitialCondition=[0 0 0]  SampleTime=Ts
  tau : Outport
  err_R : Outport  Port=2
  err_W : Outport  Port=3
  wires:
  Inner-loop control/2(omega_bb_des) -> Derivation1/1
  Inner-loop control/1(Rb_des) -> Derivation/1
  omega_bb/1 -> Inner-loop control/4(omega_bb)
  zb_des/1 -> Inner-loop control/1(zb_des)
  Derivation/1 -> Unit Delay1/1
  Unit Delay3/1 -> Inner-loop control/5(dot_omega_bb_des)
  Inner-loop control/5(err_W) -> err_W/1
  Derivation1/1 -> Unit Delay3/1
  Unit Delay1/1 -> Inner-loop control/3(dot_Rb_des)
  Inner-loop control/3(tau) -> tau/1
  Rb/1 -> Inner-loop control/2(Rb)
  Inner-loop control/4(err_R) -> err_R/1
  xb_des/1 -> Inner-loop control/6(xb_des)

== system Drone_swarm_control/Subsystem1/Subsystem_5/Planner ==
  References : Inport
  Constant : Constant  Value=0
  Demux : Demux  Outputs=10
  Mux{1..4} (4 alike) : Mux  Inputs=3
  Trigonometric Function : Trigonometry
  Trigonometric Function1 : Trigonometry  Operator=cos
  position_des : Outport
  linear_velocity_des : Outport  Port=2
  linear_acceleration_des : Outport  Port=3
  xb_des : Outport  Port=4
  wires:
  References/1 -> Demux/1
  Demux/10 -> Trigonometric Function1/1, Trigonometric Function/1
  Demux/9 -> Mux1/3
  Demux/8 -> Mux1/2
  Demux/7 -> Mux1/1
  Demux/6 -> Mux3/3
  Demux/5 -> Mux3/2
  Demux/4 -> Mux3/1
  Demux/3 -> Mux2/3
  Demux/2 -> Mux2/2
  Demux/1 -> Mux2/1
  Constant/1 -> Mux4/3
  Trigonometric Function1/1 -> Mux4/1
  Trigonometric Function/1 -> Mux4/2
  Mux4/1 -> xb_des/1
  Mux2/1 -> position_des/1
  Mux1/1 -> linear_acceleration_des/1
  Mux3/1 -> linear_velocity_des/1

== system Drone_swarm_control/Subsystem1/Subsystem_5/Quadrotor dynamics ==
  uT : Inport
  tau_b : Inport  Port=2
  Integrator : Integrator  InitialCondition=init_4
  Integrator1 : Integrator  InitialCondition=lin_vel_0
  Integrator2 : Integrator  InitialCondition=[1 0 0; 0 1 0;0 0 1]
  Integrator3 : Integrator  InitialCondition=w_bb_0
  MATLAB Function1 : MATLAB Function  TreatAsAtomicUnit=on
  UAV dynamics : MATLAB Function  TreatAsAtomicUnit=on
  Position : Outport
  Linear_velocity : Outport  Port=2
  Rb : Outport  Port=3
  dot_Rb : Outport  Port=4
  omega_bb : Outport  Port=5
  dot_omega_bb : Outport  Port=6
  lin_acc : Outport  Port=7
  wires:
  Integrator2/1 -> MATLAB Function1/1(Rb_temp)
  MATLAB Function1/1(Rb) -> UAV dynamics/3(Rb), Rb/1
  UAV dynamics/2(dot_Rb) -> dot_Rb/1, Integrator2/1
  Integrator3/1 -> omega_bb/1, UAV dynamics/4(omega_bb)
  Integrator1/1 -> Integrator/1, Linear_velocity/1
  uT/1 -> UAV dynamics/1(uT)
  UAV dynamics/1(lin_acc) -> Integrator1/1, lin_acc/1
  UAV dynamics/3(ang_acc) -> Integrator3/1, dot_omega_bb/1
  Integrator/1 -> Position/1
  tau_b/1 -> UAV dynamics/2(tau_b)

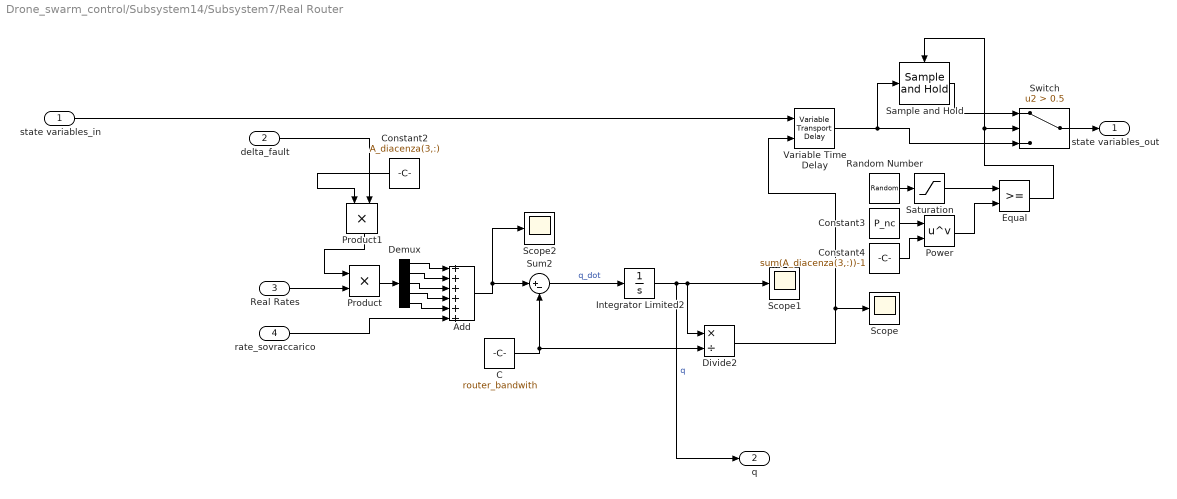
== system Drone_swarm_control/Subsystem14/Subsystem7/Real Router  ==
  state variables_in : Inport
  delta_fault : Inport  Port=2
  Real Rates : Inport  Port=3
  "rate_sovraccarico " : Inport  Port=4
  Add : Sum  Inputs=++++++
  C : Constant  Value=router_bandwith
  Constant2 : Constant  Value=A_diacenza(3,:)
  Constant3 : Constant  Value=P_nc
  Constant4 : Constant  Value=sum(A_diacenza(3,:))-1
  Demux : Demux  Outputs=5
  Divide2 : Product  Inputs=*/
  Equal : RelationalOperator  OutDataTypeStr=boolean  RndMeth=Simplest  InputSameDT=off
  Integrator Limited2 : Integrator  InitialCondition=router_init_queue(3)  LimitOutput=on  UpperSaturationLimit=router_buffer  LowerSaturationLimit=0
  Power : Math  Operator=pow
  Product : Product
  Product1 : Product
  Random Number : RandomNumber  Mean=0.5  Variance=0.5  SampleTime=0.1
  Sample and Hold : dspsigops/Sample and Hold  trig=Rising edge  initCond=0  latchinput=off
  Saturation : Saturate  UpperLimit=1  LowerLimit=0
  Scope : Scope
      settings: ActiveDisplayYMinimum=-1  ActiveDisplayYMaximum=1  DataLoggingVariableName=ScopeData7
  Scope1 : Scope
      settings: ActiveDisplayYMinimum=1.4313918245472816  ActiveDisplayYMaximum=3.3975685911844873  DataLoggingVariableName=ScopeData8
  Scope2 : Scope
      settings: ActiveDisplayYMinimum=-5.0715881779365786  ActiveDisplayYMaximum=37.614274886734989  DataLoggingVariableName=ScopeData23
  Sum2 : Sum  Inputs=|+-
  Switch : Switch  Criteria=u2 > Threshold  Threshold=0.5  SaturateOnIntegerOverflow=off  InputSameDT=off
  Variable Time Delay : VariableTransportDelay  MaximumDelay=1000  InitialOutput=[init_0;zeros(6,1);init_1;zeros(6,1);init_2;zeros(6,1);init_3;zeros(6,1);init_4;zeros(6,1);]  MaximumPoints=1e4  ZeroDelay=on
  state variables_out : Outport
  q : Outport  Port=2
  wires:
  Demux/2 -> Add/2
  Variable Time Delay/1 -> Sample and Hold/1, Switch/3
  Add/1 -> Scope2/1, Sum2/1
  Constant3/1 -> Power/1
  Product/1 -> Demux/1
  Constant4/1 -> Power/2
  Product1/1 -> Product/1
  Demux/3 -> Add/3
  Power/1 -> Equal/2
  Equal/1 -> Switch/2, Sample and Hold/Trigger
  Sum2/1 -> Integrator Limited2/1  "q_dot"
  Saturation/1 -> Equal/1
  Integrator Limited2/1 -> q/1, Scope1/1, Divide2/1  "q"
  Switch/1 -> state variables_out/1
  Divide2/1 -> Scope/1, Variable Time Delay/2
  Demux/1 -> Add/1
  Constant2/1 -> Product1/1
  Demux/4 -> Add/4
  Random Number/1 -> Saturation/1
  delta_fault/1 -> Product1/2
  Sample and Hold/1 -> Switch/1
  C/1 -> Divide2/2, Sum2/2
  Demux/5 -> Add/5
  state variables_in/1 -> Variable Time Delay/1
  Real Rates/1 -> Product/2
  "rate_sovraccarico "/1 -> Add/6

== system Drone_swarm_control/Subsystem14/Subsystem7/virtual router ==
  q_ref : Inport
  C1 : Constant  Value=router_bandwith*0.8
  Integrator Limited1 : Integrator  InitialCondition=router_init_queue(1)  LimitOutput=on  UpperSaturationLimit=router_buffer  LowerSaturationLimit=0
  PID Controller : slpidlib/PID Controller  Controller=PID  Form=Parallel  TimeDomain=Continuous-time  UseExternalTs=off  SampleTime=-1  IntegratorMethod=Forward Euler  FilterMethod=Forward Euler  ControllerParametersSource=internal  P=PID_p  I=PID_i  UseKiTs=off  D=PID_d  UseExternalDerivativeSource=off  N=100  UseFilter=on  TunerSelectOption=Transfer Function Based (PID Tuner App)  InitialConditionSource=internal  InitialConditionForIntegrator=0  InitialConditionForFilter=0  DifferentiatorICPrevScaledInput=0  ExternalReset=none  TrackingMode=off  Kt=1  LimitOutput=off  SatLimitsSource=internal  UpperSaturationLimit=inf  LowerSaturationLimit=-inf  LinearizeAsGain=on  AntiWindupMode=none  Kb=1  LimitIntegrator=off  UpperIntegratorSaturationLimit=inf  LowerIntegratorSaturationLimit=-inf  POutMin=[]  POutMax=[]  IOutMin=[]  IOutMax=[]  DOutMin=[]  DOutMax=[]  NOutMin=[]  NOutMax=[]  SumOutMin=[]  SumOutMax=[]  SaturationOutMin=[]  SaturationOutMax=[]  PParamMin=[]  PParamMax=[]  IParamMin=[]  IParamMax=[]  DParamMin=[]  DParamMax=[]  NParamMin=[]  NParamMax=[]  KbParamMin=[]  KbParamMax=[]  KtParamMin=[]  KtParamMax=[]  KbOutMin=[]  KbOutMax=[]  KtOutMin=[]  KtOutMax=[]  IntegratorOutMin=[]  IntegratorOutMax=[]  FilterOutMin=[]  FilterOutMax=[]  SumI1OutMin=[]  SumI1OutMax=[]  SumI2OutMin=[]  SumI2OutMax=[]  SumI3OutMin=[]  SumI3OutMax=[]  SumI4OutMin=[]  SumI4OutMax=[]  SumDOutMin=[]  SumDOutMax=[]  DifferentiatorOutMin=[]  DifferentiatorOutMax=[]  FilterDiffOutCoefMin=[]  FilterDiffOutCoefMax=[]  ReciprocalOutMin=[]  ReciprocalOutMax=[]  SumDenOutMin=[]  SumDenOutMax=[]  SumNumOutMin=[]  SumNumOutMax=[]  DivideOutMin=[]  DivideOutMax=[]  UdiffTsProdOutMin=[]  UdiffTsProdOutMax=[]  NTsProdOutMin=[]  NTsProdOutMax=[]  UintegralTsProdOutMin=[]  UintegralTsProdOutMax=[]  UngainTsProdOutMin=[]  UngainTsProdOutMax=[]  ClampingZeroOutDataTypeStr=Inherit: Inherit via back propagation  ClampingZeroOutMin=[]  ClampingZeroOutMax=[]  FilterDenConstantOutDataTypeStr=Inherit: Inherit via back propagation  FilterDenConstantOutMin=[]  FilterDenConstantOutMax=[]  PCopyOutDataTypeStr=Inherit: Inherit via back propagation  PCopyOutMin=[]  PCopyOutMax=[]  NCopyOutDataTypeStr=Inherit: Inherit via back propagation  NCopyOutMin=[]  NCopyOutMax=[]  IntegratorContinuousStateAttributes=''  IntegratorStateMustResolveToSignalObject=off  IntegratorRTWStateStorageClass=Auto  FilterContinuousStateAttributes=''  FilterStateMustResolveToSignalObject=off  FilterRTWStateStorageClass=Auto  ParallelPVariant=InternalParameters  IdealPVariant=Disabled  IVariant=InternalParameters  DVariant=InternalParameters  IntegratorVariant=Continuous  SatVariant=Disabled  AWVariant=Passthrough  PCopyVariant=Disabled  TRVariant=Disabled  FdbkBlocksVariant=Forward  IdealPFdbkVariant=Disabled  SatFdbkVariant=Disabled  DerivativeFilterVariant=ContFilter  NVariant=InternalParameters  NCopyVariant=Disabled  FilterICVariant=InternalICsFilter  IntegratorICVariant=InternalICs  ExternalResetVariant=Disabled  TRSumVariant=Passthrough  SumFdbkVariant=Disabled  SumVariant=Sum_PID  TsampFilterVariant=InternalTs  TsampNgainVariant=Passthrough  TsampIntegralVariant=Disabled_SignalSpec  ExternalSaturationOutDataTypeStr=Inherit: Same as second input  DerivativeSourceVariant=ErrorSignal  PreIntVariant=InternalPreInt
  Scope3 : Scope
      settings: ActiveDisplayYMinimum=18.031914924971169  ActiveDisplayYMaximum=21.223404282118214  DataLoggingVariableName=ScopeData18
  Scope4 : Scope
      settings: ActiveDisplayYMinimum=-3.625  ActiveDisplayYMaximum=2.625  DataLoggingVariableName=ScopeData19
  Sum : Sum  Inputs=|+-
  Sum1 : Sum  Inputs=|+-
  r_req : Outport
  wires:
  Sum/1 -> Scope4/1, PID Controller/1
  Sum1/1 -> Integrator Limited1/1  "q_dot"
  PID Controller/1 -> Sum1/1, r_req/1, Scope3/1
  Integrator Limited1/1 -> Sum/2  "q"
  C1/1 -> Sum1/2
  q_ref/1 -> Sum/1

== matlab function Drone_swarm_control/trasmission/rate_min/MATLAB Function2 ==
  data: u input; y output
function y = fcn(u)
% Handle inactive channels before selecting a communication rate.


for i=1:5
    if u(i)==0
        u(i)=1000;
    end
end

% Reset the output when the minimum equals the fallback value.
if min(u)==1000
    u=zeros(5,1);
end
y = u;

end

== matlab function Drone_swarm_control/trasmission/rate_min/MATLAB Function3 ==
  data: u input; y output
function y = fcn(u)
% Handle inactive channels before selecting a communication rate.


for i=1:5
    if u(i)==0
        u(i)=1000;
    end
end

% Reset the output when the minimum equals the fallback value.
if min(u)==1000
    u=zeros(5,1);
end
y = u;

end

== matlab function Drone_swarm_control/trasmission/rate_min/MATLAB Function4 ==
  data: u input; y output
function y = fcn(u)
% Handle inactive channels before selecting a communication rate.


for i=1:5
    if u(i)==0
        u(i)=1000;
    end
end

% Reset the output when the minimum equals the fallback value.
if min(u)==1000
    u=zeros(5,1);
end
y = u;

end

== matlab function Drone_swarm_control/Subsystem11/MATLAB Function1 ==
  data: A input; K_edit output; delta input; i input
function K_edit = fcn(A,delta,i)
% Rebuild the selected coupling row using the node-availability mask.



A_edit=A(i,:);

A_edit=delta&apos;.*A_edit;

D = diag(sum(A_edit&apos;));
L = -A_edit;
L(i)=D-L(i);
I_9 = eye(9);
K_edit = kron(L,I_9);
% Disable the coupling term when the node is inactive.
if delta(i)==0
    K_edit = zeros(9,45);
end
end

== matlab function Drone_swarm_control/Subsystem11/MATLAB Function2 ==
  data: A input; K_edit output; delta input; i input
function K_edit = fcn(A,delta,i)
% Rebuild the selected coupling row using the node-availability mask.



A_edit=A(i,:);

A_edit=delta&apos;.*A_edit;

D = diag(sum(A_edit&apos;));
L = -A_edit;
L(i)=D-L(i);
I_9 = eye(9);
K_edit = kron(L,I_9);
% Disable the coupling term when the node is inactive.
if delta(i)==0
    K_edit = zeros(9,45);
end
end

== matlab function Drone_swarm_control/Subsystem11/MATLAB Function3 ==
  data: A input; K_edit output; delta input; i input
function K_edit = fcn(A,delta,i)
% Rebuild the selected coupling row using the node-availability mask.



A_edit=A(i,:);

A_edit=delta&apos;.*A_edit;

D = diag(sum(A_edit&apos;));
L = -A_edit;
L(i)=D-L(i);
I_9 = eye(9);
K_edit = kron(L,I_9);
% Disable the coupling term when the node is inactive.
if delta(i)==0
    K_edit = zeros(9,45);
end
end

== matlab function Drone_swarm_control/Subsystem11/MATLAB Function4 ==
  data: A input; K_edit output; delta input; i input
function K_edit = fcn(A,delta,i)
% Rebuild the selected coupling row using the node-availability mask.



A_edit=A(i,:);

A_edit=delta&apos;.*A_edit;

D = diag(sum(A_edit&apos;));
L = -A_edit;
L(i)=D-L(i);
I_9 = eye(9);
K_edit = kron(L,I_9);
% Disable the coupling term when the node is inactive.
if delta(i)==0
    K_edit = zeros(9,45);
end
end

== matlab function Drone_swarm_control/trasmission/MATLAB Function5 ==
  data: A input; y output; delta_fault input
function y = fcn(A,delta_fault)
% Normalize communication links after excluding inactive nodes.

A_edit=diag(delta_fault)*A*diag(delta_fault);
y_=1./(sum(A_edit&apos;)+(ones(1,5)-delta_fault&apos;)+[1,0,0,0,0]);

y=y_&apos;;


end

== matlab function Drone_swarm_control/Subsystem11/MATLAB Function6 ==
  data: A input; K_edit output; delta input; i input
function K_edit = fcn(A,delta,i)
% Rebuild the selected coupling row using the node-availability mask.



A_edit=A(i,:);

A_edit=delta&apos;.*A_edit;

D = diag(sum(A_edit&apos;));
L_edit = -A_edit;
L_edit(i)=D-L_edit(i);
I_9 = eye(9);
K_edit = kron(L_edit,I_9);

% Disable the coupling term when the node is inactive.
if delta(i)==0
    K_edit = zeros(9,45);
end

end

== matlab function Drone_swarm_control/trasmission/rate_min/MATLAB Function5 ==
  data: A input; A_edit1 output; delta input; A_edit2 output; A_edit3 output; A_edit4 output; A_edit5 output
function [A_edit1,A_edit2,A_edit3,A_edit4,A_edit5] = fcn(A,delta)
% Mask incoming and outgoing communication links for each drone.

A_edit1=A(:,1);
A_edit1=delta.*A_edit1*delta(1);

A_edit2=A(:,2);
A_edit2=delta.*A_edit2*delta(2);

A_edit3=A(:,3);
A_edit3=delta.*A_edit3*delta(3);

A_edit4=A(:,4);
A_edit4=delta.*A_edit4*delta(4);

A_edit5=A(:,5);
A_edit5=delta.*A_edit5*delta(5);



end

== matlab function Drone_swarm_control/Subsystem1/Subsystem_1/Quadrotor dynamics/UAV dynamics ==
  data: uT input size=1; tau_b input size=3; lin_acc output size=3; Rb input size=[3,3]; omega_bb input size=3; dot_Rb output size=[3,3]; ang_acc output size=3; mass parameter size=1; Ib parameter size=[3,3]
function [lin_acc, dot_Rb, ang_acc] = fcn(uT,tau_b,Rb,omega_bb,mass, Ib)
% Quadrotor translational and rotational rigid-body dynamics.

lin_acc = 9.81*[0 0 1]&apos;-(uT/mass)*Rb*[0 0 1]&apos;;
dot_Rb = Rb*skew(omega_bb);
ang_acc = inv(Ib)*(-skew(omega_bb)*Ib*omega_bb + tau_b);

end

function S = skew(v)
% Matrix representation of the cross product.
if(numel(v)~= 1)
S= [0 -v(3) v(2); 
    v(3) 0 -v(1);
    -v(2) v(1) 0];
else
S= zeros(3);
end
end

== matlab function Drone_swarm_control/Subsystem7/MATLAB Function ==
  data: v input; P output; a input; f input; E input; E_new output
function [P, E_new] = batteryDischargeXYZ(v, a, f, E)
% Estimate instantaneous power and update the remaining battery energy.

P_base = 130;
k_v = 0.69;
k_a = 10;
k_f = 0.001;

v_mag = norm(v);
a_mag = norm(a);

% Combine hovering, motion and packet-transmission power.
P = P_base + k_v * v_mag^2 + k_a * a_mag + k_f * f;

% Energy decrement using the existing 1 ms update step.
dE_dt = 0.001*(-P / 3600);

% Stop the decrement after battery depletion.
if E <= 0
    dE_dt = 0;
end

E_new=E+dE_dt;
end

== matlab function Drone_swarm_control/MATLAB Function2 ==
  data: M input; vec output; V input; A input
function vec = concatena_colonne(M, V, A)
% Stack state columns for the network controller.
    C = zeros(3, 15);

    C(:, 1:3:end) = M;
    C(:, 2:3:end) = V;
    C(:, 3:3:end) = A;

    vec = C(:);
end

== matlab function Drone_swarm_control/Subsystem7/MATLAB Function1 ==
  data: v input; P output; a input; f input; E input; E_new output
function [P, E_new] = batteryDischargeXYZ(v, a, f, E)
% Estimate instantaneous power and update the remaining battery energy.

P_base = 130;
k_v = 0.69;
k_a = 10;
k_f = 0.001;

v_mag = norm(v);
a_mag = norm(a);

% Combine hovering, motion and packet-transmission power.
P = P_base + k_v * v_mag^2 + k_a * a_mag + k_f * f;

% Energy decrement using the existing 1 ms update step.
dE_dt = 0.001*(-P / 3600);

% Stop the decrement after battery depletion.
if E <= 0
    dE_dt = 0;
end

E_new=E+dE_dt;
end
